simulink model "MPPT_4x4"  (R2025b)
settings: Solver=ode23t  StartTime=0.0  StopTime=Tstop  MaxStep=1e-4  RelTol=1e-3
model workspace (MAT data in the model file):
  Cin = 0.00022
  Cin_esr = 0.05
  Cout = 0.00047
  G_tau = 0.001
  Gsched = [0 1000 1000 1000 1000 1000 1000 1000 1000 1000 1000 1000 ... (17 elements, 1x17)]
  L = 0.00015
  RL = 0.01
  Rc = 0.05
  Rload = 10
  Tlog = 0.0005
  Tstop = 2
  byp_Goff = 4.4e-06
  byp_Ron = 0.012
  byp_Vf = 0.37
  mppt : object (value not decoded)
  pv_Ir0 = 1000
  pv_Isc = 9.11
  pv_Ncell = 72
  pv_Ngrp = 24
  pv_Rs = 0.00441
  pv_Voc = 0.636111111111
  pv_n = 1
symbols that are objects in the model workspace (value not decoded): mppt
libraries: ee_lib x97, nesl_utility x21, fl_lib x6
(part 4 of 4)

== matlab function MPPT_4x4/Controller/MPPT ==
  settings: updateMethod=DISCRETE  sampleTime=mppt.Tc
  data: Vpv input; D output; Ipv input; Vm output; Im output; mppt parameter
function [D, Vm, Im] = MPPT(Vpv, Ipv, mppt)
% One call per control sample. The algorithm is in mppt_controller.m.
[D, Vm, Im] = mppt_controller(Vpv, Ipv, mppt);
